simulink model "sm_car_"  (R2026b)
settings: Solver=ode23t  StopTime=100  MaxStep=0.4  AbsTol=1e-3  EnableMultiTasking=on
PreLoadFcn:
  | % Due to usability issue in Repeating Sequence block
  | warning('off','Simulink:Masking:Invalid');
  | 
  | % Eliminate unnecessary warnings in inactive variants
  | % Warnings generated only if you click through inactive variant
  | warning('off','MATLAB:nonExistentField');
  | warning('off','Simulink:Parameters:BlkParamUndefined');
PostLoadFcn:
  | set_param([bdroot '/Vehicle'],'popup_trailer','Off')
  | warning('off','sm:sli:setup:compile:LocalSolverNotSupported')
  | %sm_car_config_maneuver(bdroot,'WOT Braking');
  | sm_car_config_vehicle(bdroot,'false');
  | sm_car_config_logging(bdroot);
InitFcn:
  | sm_car_config_camera;
  | Vehicle = sm_car_vehcfg_checkConfig(Vehicle);
  | sm_car_check_tire_model(bdroot);
StartFcn:
  | tic;
StopFcn:
  | Elapsed_Sim_Time = toc;
  | % disp(['Elapsed Sim Time = ' num2str(Elapsed_Sim_Time)]);
undefined symbols (not defined in the file or in its folder): acc_theta, accel_ramp_rate, Axle1D, AxleIn, Camera, Control, Driver, Init, Maneuver, Pedal, Scene, ShaftL1, ShaftL2, ShaftR1, ShaftR2, Visual, X, xy_data_car_side, Y, Z
libraries: sm_lib x290, fl_lib x171, nesl_utility x144, simulink x60, simulink_extras x14, sdl_lib x14, SimscapeFluids_lib x7, Damper_Element x4, Tire_1x2x x4, ee_lib x3, Scene_Utilities x3, sharedTrackingLibrary x2
(part 9 of 22)

== system sm_car_/Controller/TrqVec_FLC/Brake Control/Pedal ==
  rBrakePedal : Inport
  VehBus : Inport  Port=2
  Apply{,1..3} (4 alike) : Constant  Value=[0 1]
  Bus Creator : BusCreator  Inputs=1
  Bus Creator1 : BusCreator  Inputs=4
  Terminator : Terminator
  Terminator1 : Terminator
  Brakes : Outport  VectorParamsAs1DForOutWhenUnconnected=off
  wires:
  rBrakePedal/1 -> Terminator1/1
  Apply3/1 -> Bus Creator1/4  "R2"
  Apply2/1 -> Bus Creator1/3  "L2"
  Apply1/1 -> Bus Creator1/2  "R1"
  Apply/1 -> Bus Creator1/1  "L1"
  Bus Creator1/1 -> Bus Creator/1  "Valves"
  VehBus/1 -> Terminator/1
  Bus Creator/1 -> Brakes/1  "Brakes"

== system sm_car_/Controller/TrqVec_FLC_V2/Brake Control/Pedal ==
  rBrakePedal : Inport
  VehBus : Inport  Port=2
  Apply{,1..3} (4 alike) : Constant  Value=[0 1]
  Bus Creator : BusCreator  Inputs=1
  Bus Creator1 : BusCreator  Inputs=4
  Terminator : Terminator
  Terminator1 : Terminator
  Brakes : Outport  VectorParamsAs1DForOutWhenUnconnected=off
  wires:
  Bus Creator/1 -> Brakes/1  "Brakes"
  VehBus/1 -> Terminator/1
  Bus Creator1/1 -> Bus Creator/1  "Valves"
  Apply/1 -> Bus Creator1/1  "L1"
  Apply1/1 -> Bus Creator1/2  "R1"
  Apply2/1 -> Bus Creator1/3  "L2"
  Apply3/1 -> Bus Creator1/4  "R2"
  rBrakePedal/1 -> Terminator1/1

== system sm_car_/Controller/TrqVec_FLC_V3/Brake Control/Pedal ==
  rBrakePedal : Inport
  VehBus : Inport  Port=2
  Apply{,1..3} (4 alike) : Constant  Value=[0 1]
  Bus Creator : BusCreator  Inputs=1
  Bus Creator1 : BusCreator  Inputs=4
  Terminator : Terminator
  Terminator1 : Terminator
  Brakes : Outport  VectorParamsAs1DForOutWhenUnconnected=off
  wires:
  rBrakePedal/1 -> Terminator1/1
  Apply3/1 -> Bus Creator1/4  "R2"
  Apply2/1 -> Bus Creator1/3  "L2"
  Apply1/1 -> Bus Creator1/2  "R1"
  Apply/1 -> Bus Creator1/1  "L1"
  Bus Creator1/1 -> Bus Creator/1  "Valves"
  VehBus/1 -> Terminator/1
  Bus Creator/1 -> Brakes/1  "Brakes"

== system sm_car_/Controller/TrqVec_FLC_V3/Power Control/State Estimation ==
  aSteerWheel : Inport
  VehBus : Inport  Port=2
  Bus Creator : BusCreator  Inputs=5
  Bus Selector : BusSelector  OutputSignals=World.vx,World.vy,World.vz,Chassis.Body.CG.nYaw,Chassis.Body.CG.gx,Chassis.Body.CG.gy,Chassis.SuspA1.LinkageL.Upright.Upright.w,Chassis.SuspA1.LinkageR.Upright.Upright.w,Chassis.SuspA2.LinkageL.Upright.Upright.w,Chassis.SuspA2.LinkageR.Upright.Upright.w
  Data Type Conversion : DataTypeConversion  OutDataTypeStr=double  SaturateOnIntegerOverflow=off  RndMeth=Floor
  Data Type Conversion1 : DataTypeConversion  OutDataTypeStr=double  SaturateOnIntegerOverflow=off  RndMeth=Floor
  Demux : Demux  Outputs=5
  Rate Transition1 : RateTransition  Deterministic=off  OutPortSampleTime=0.003
  Rate Transition2 : RateTransition  Deterministic=off  OutPortSampleTime=0.003
  Rate Transition4 : RateTransition  Deterministic=off
  Sensor Noise Simulation : Subsystem
  UKF : Subsystem
  StateEst : Outport
  Out Bus Element : Outport  Port=2  PortName=Meas  Element=Meas
  Out Bus Element1 : Outport  Port=2  PortName=Meas  Element=Input
  Out Bus Element2 : Outport  Port=2  PortName=Meas  Element=State
  wires:
  Bus Selector/3 -> Sensor Noise Simulation/3(<vz>)  "<vz>"
  Rate Transition4/1 -> Out Bus Element1/1
  Data Type Conversion1/1 -> Rate Transition4/1
  UKF/1(xhat) -> Data Type Conversion/1
  Rate Transition2/1 -> UKF/2(y1)
  Rate Transition1/1 -> UKF/1(StateTransitionFcnInputs)
  Demux/5 -> Bus Creator/5  "a_y"
  Demux/4 -> Bus Creator/4  "a_x"
  Demux/3 -> Bus Creator/3  "phi_dot"
  Demux/2 -> Bus Creator/2  "v_y"
  Demux/1 -> Bus Creator/1  "v_x"
  Bus Creator/1 -> StateEst/1, Out Bus Element2/1  "UKF"
  Data Type Conversion/1 -> Demux/1
  Sensor Noise Simulation/1(Inputs) -> Rate Transition1/1, Data Type Conversion1/1  "Input"
  Sensor Noise Simulation/2(Meas) -> Out Bus Element/1, Rate Transition2/1  "Measument"
  aSteerWheel/1 -> Sensor Noise Simulation/11(delta)  "delta"
  Bus Selector/10 -> Sensor Noise Simulation/10(<w_rr>)  "<w>"
  Bus Selector/9 -> Sensor Noise Simulation/9(<w_rl>)  "<w>"
  Bus Selector/8 -> Sensor Noise Simulation/8(<w_fr>)  "<w>"
  Bus Selector/7 -> Sensor Noise Simulation/7(<w_fl>)  "<w>"
  Bus Selector/6 -> Sensor Noise Simulation/6(<gy>)  "<gy>"
  Bus Selector/5 -> Sensor Noise Simulation/5(<gx>)  "<gx>"
  Bus Selector/4 -> Sensor Noise Simulation/4(<nYaw>)  "<nYaw>"
  Bus Selector/2 -> Sensor Noise Simulation/2(<vy>)  "<vy>"
  Bus Selector/1 -> Sensor Noise Simulation/1(<vx>)  "<vx>"
  VehBus/1 -> Bus Selector/1

== system sm_car_/Driver/Closed Loop/Driver/Get Pose ==
  Ref : Inport
  Bus Selector : BusSelector  OutputSignals=x,y,ayaw
  Gain : Gain  Gain=180/pi
  Mux : Mux  Inputs=3
  RefPose : Outport  VectorParamsAs1DForOutWhenUnconnected=off
  wires:
  Gain/1 -> Mux/3
  Bus Selector/3 -> Gain/1  "<ayaw>"
  Bus Selector/2 -> Mux/2  "<y>"
  Mux/1 -> RefPose/1
  Ref/1 -> Bus Selector/1
  Bus Selector/1 -> Mux/1  "<x>"

== system sm_car_/Driver/Closed Loop/Driver Override/None ==
  In : Inport
  DrvBus : Outport
  wires:
  In/1 -> DrvBus/1

== system sm_car_/Driver/Closed Loop/Driver Override/Override ==
  In : Inport
  Bus Creator5 : BusCreator  Inputs=4
  Bus Selector : BusSelector  OutputSignals=Reference,aSteerWheel,rAccelPedal,rBrakePedal
  Clock : Clock
  Compare To Constant : simulink/Logic and Bit Operations/Compare To Constant  relop=>=  const=Maneuver.TStart.aSteer.Value  OutDataTypeStr=boolean
  Compare To Constant1 : simulink/Logic and Bit Operations/Compare To Constant  relop=>=  const=Maneuver.TStart.rAccel.Value  OutDataTypeStr=boolean
  Compare To Constant2 : simulink/Logic and Bit Operations/Compare To Constant  relop=>=  const=Maneuver.TStart.rBrake.Value  OutDataTypeStr=boolean
  Input Sequence Accel Pedal : simulink/Sources/Repeating Sequence  rep_seq_t=Maneuver.Accel.t.Value  rep_seq_y=Maneuver.Accel.rPedal.Value
  Input Sequence Brake Pedal : simulink/Sources/Repeating Sequence  rep_seq_t=Maneuver.Brake.t.Value  rep_seq_y=Maneuver.Brake.rPedal.Value
  Input Sequence Steering Wheel : simulink/Sources/Repeating Sequence  rep_seq_t=Maneuver.Steer.t.Value  rep_seq_y=Maneuver.Steer.aWheel.Value
  Switch : Switch  Criteria=u2 > Threshold  SaturateOnIntegerOverflow=off  InputSameDT=off
  Switch1 : Switch  Criteria=u2 > Threshold  SaturateOnIntegerOverflow=off  InputSameDT=off
  Switch2 : Switch  Criteria=u2 > Threshold  SaturateOnIntegerOverflow=off  InputSameDT=off
  DrvBus : Outport
  wires:
  Input Sequence Brake Pedal/1 -> Switch2/1  "rBrakePedal"
  Input Sequence Accel Pedal/1 -> Switch1/1  "rAccelPedal"
  Input Sequence Steering Wheel/1 -> Switch/1  "aSteerWheel"
  Switch2/1 -> Bus Creator5/4  "rBrakePedal"
  Compare To Constant/1 -> Switch/2
  Clock/1 -> Compare To Constant/1, Compare To Constant1/1, Compare To Constant2/1
  Bus Selector/4 -> Switch2/3  "<rBrakePedal>"
  Switch1/1 -> Bus Creator5/3  "rAccelPedal"
  Bus Selector/3 -> Switch1/3  "<rAccelPedal>"
  Bus Selector/1 -> Bus Creator5/1  "<Reference>"
  Switch/1 -> Bus Creator5/2  "aSteerWheel"
  Bus Selector/2 -> Switch/3  "<aSteerWheel>"
  Bus Creator5/1 -> DrvBus/1  "DrvBus"
  In/1 -> Bus Selector/1
  Compare To Constant1/1 -> Switch1/2
  Compare To Constant2/1 -> Switch2/2

== system sm_car_/Driver/Closed Loop/Maneuver/Count Lap ==
  note: If on the previous step, the vehicle was in the first 5 percent of the trajectory and now it is on the last 5 percent of the trajectory, decrement the number of laps.
  note: If on the previous step, the vehicle was in the last 5 percent of the trajectory and now it is on the first 5 percent of the trajectory, increment the number of laps.
  ad : Inport
  AND Add Lap : Logic  IconShape=distinctive  AllPortsSameDT=off  OutDataTypeStr=boolean
  AND Subtract Lap : Logic  IconShape=distinctive  AllPortsSameDT=off  OutDataTypeStr=boolean
  Data Type Conversion : DataTypeConversion  SaturateOnIntegerOverflow=off  RndMeth=Floor
  Data Type Conversion1 : DataTypeConversion  SaturateOnIntegerOverflow=off  RndMeth=Floor
  First 5 Percent : simulink/Logic and Bit Operations/Compare To Constant  relop=<=  const=max(Maneuver.Trajectory.xTrajectory.Value)*0.05  OutDataTypeStr=boolean  ZeroCross=off
  Last 5 Percent : simulink/Logic and Bit Operations/Compare To Constant  relop=>=  const=max(Maneuver.Trajectory.xTrajectory.Value)*0.95  OutDataTypeStr=boolean  ZeroCross=off
  Memory : Memory  InitialCondition=false
  Memory2 : Memory  InitialCondition=false
  OR : Logic  Operator=OR  IconShape=distinctive  AllPortsSameDT=off  OutDataTypeStr=boolean
  Sum : Sum  Inputs=+-|
  Triggered Subsystem : Subsystem  TreatAsAtomicUnit=on
  lapC : Outport  VectorParamsAs1DForOutWhenUnconnected=off
  wires:
  Sum/1 -> Triggered Subsystem/1(Up Down)  "Counter"
  AND Subtract Lap/1 -> Data Type Conversion1/1, OR/2  "Subtract Lap"
  AND Add Lap/1 -> OR/1, Data Type Conversion/1  "Add Lap"
  Memory2/1 -> AND Subtract Lap/1
  OR/1 -> Triggered Subsystem/Trigger  "Trigger"
  Memory/1 -> AND Add Lap/1
  First 5 Percent/1 -> AND Add Lap/2, Memory2/1  "First 5"
  Triggered Subsystem/1(Num Laps) -> lapC/1
  Last 5 Percent/1 -> Memory/1, AND Subtract Lap/2  "Last 5"
  ad/1 -> Last 5 Percent/1, First 5 Percent/1
  Data Type Conversion/1 -> Sum/1
  Data Type Conversion1/1 -> Sum/2

== system sm_car_/Driver/Closed Loop/Maneuver/PoseTargetVisual ==
  note: Allow yaw angle to wrap for
      | clockwise and counterclockwise laps.
  dist : Inport
  ref_x : Inport  Port=2
  ref_y : Inport  Port=3
  ref_z : Inport  Port=4
  ref_ayaw : Inport  Port=5
  CW or CCW : Constant  Value=sign(Maneuver.Trajectory.aYaw.Value(end)-Maneuver.Trajectory.aYaw.Value(1))
  Count Lap : Subsystem
  Gain : Gain  Gain=2*pi
  MechanismConfiguration : sm_lib/Utilities/Mechanism Configuration  UniformGravity=None  GravityVector=[0 0 -9.80665]  GravityVectorUnits=m/s^2  LinearizationDelta=0.001  JointModeTransitionNonlinearIterations=2
  Pace Car : Subsystem  mask(Car Body Geometry){whl_cutout_rad=0.5, whl_base=abs(Vehicle.Chassis.Body.sAxle1.Value(1)-Vehicle.Chassis.Body.sAxle2.Value(1)), thk_top=0.05, thk_side=0.05, car_track=Vehicle.Chassis.Body.Width.Value, offset_ref=[0 0 0.3225], extr_data_emblem_f=Visual.PaceCar.emblem.data*0.2, extr_data_emblem_r=Visual.PaceCar.emblem.data*0.2, clr_body_geo_top=Visual.PaceCar.body.clr, opc_body_geo_top=Visual.PaceCar.body.opc, clr_body_geo_left=Visual.PaceCar.body.clr, opc_body_geo_left=Visual.PaceCar.body.opc, clr_body_geo_right=Visual.PaceCar.body.clr, opc_body_geo_right=Visual.PaceCar.body.opc, clr_emblem_f=Visual.PaceCar.body.clr, opc_emblem_f=Visual.PaceCar.emblem.opc, clr_emblem_r=Visual.PaceCar.body.clr, opc_emblem_r=Visual.PaceCar.emblem.opc}
      mask prompts: whl_cutout_rad "Wheel Cutout Radius (m)"; whl_base "Wheelbase (m)"; thk_top "Top Thickness (m)"; thk_side "Side Thickness (m)"; car_track "Width (m)"; offset_ref "Offset to reference frame [xyz] (m)"; extr_data_emblem_f "Emblem Data Front [xy] (m)"; extr_data_emblem_r "Emblem Data Rear [xy] (m)"
      mask help: Creates simple car geometry. Adjusting the wheel cutout radius and wheelbase causes the profile to be adjusted. Press the Plot Profile button to see how the parameters affect the profile.
      mask init:
      | [xy_data_car_top xy_data_car_side] = Extr_Data_Car_Profile(whl_cutout_rad, whl_base,thk_top);
      mask TypeOptions extr_data_emblem_f:
      | Ornament
      | Front/ExtrusionCrossSection
      mask TypeOptions extr_data_emblem_r:
      | Ornament
      | Rear/ExtrusionCrossSection
      mask TypeOptions clr_body_geo_top: Top Surface/GraphicDiffuseColor
      mask TypeOptions opc_body_geo_top: Top Surface/GraphicOpacity
      mask TypeOptions clr_body_geo_left: Left Face/GraphicDiffuseColor
      mask TypeOptions opc_body_geo_left: Left Face/GraphicOpacity
      mask TypeOptions clr_body_geo_right: Right Face/GraphicDiffuseColor
      mask TypeOptions opc_body_geo_right: Right Face/GraphicOpacity
      mask TypeOptions clr_emblem_f:
      | Ornament
      | Front/GraphicDiffuseColor
      mask TypeOptions opc_emblem_f:
      | Ornament
      | Front/GraphicOpacity
      mask TypeOptions clr_emblem_r:
      | Ornament
      | Rear/GraphicDiffuseColor
      mask TypeOptions opc_emblem_r:
      | Ornament
      | Rear/GraphicOpacity
      mask DialogControl cont_geometry Prompt: Body Geometry
      mask DialogControl push_plot_profile Prompt: Plot Profile
      mask DialogControl push_plot_profile Callback:
      | v = get_param(gcb,'MaskWSVariables');
      | getMaskValue = containers.Map({v.Name}',{v.Value}');
      | evalin('base',...
      |     sprintf('Extr_Data_Car_Profile(%s,%s,%s,''%s'');',...
      |     num2str(getMaskValue('whl_cutout_rad')),...
      |     num2str(getMaskValue('whl_base')),...
      |     num2str(getMaskValue('thk_top')),'plot'));
      mask DialogControl cont_emblem Prompt: Emblem
      mask DialogControl cont_vis Prompt: Visualization
      mask DialogControl text_vis_clr Prompt: Color [RGB]
      mask DialogControl text_vis_opc Prompt: Opac. (0-1)
      mask DialogControl text_vis_top Prompt: Top
      mask DialogControl text_vis_left Prompt: Left Side
      mask DialogControl text_vis_right Prompt: Right Side
      mask DialogControl text_vis_emblem_f Prompt: Emblem Front
      mask DialogControl text_vis_emblem_r Prompt: Emblem Rear
      mask Display: image('sm_car_bodygeometry_sedan.png');
  Planar Joint : sm_lib/Joints/Planar Joint  JointMode=Normal  CompositeWrenchDir=FollowerOnBase  CompositeWrenchFrame=BaseFrame  SenseConstraintForce=off  SenseConstraintTorque=off  SenseTotalForce=off  SenseTotalTorque=off  PxPositionTargetSpecify=off  PxPositionTargetPriority=High  PxPositionTargetValue=0  PxPositionTargetValueUnits=m  PxVelocityTargetSpecify=off  PxVelocityTargetPriority=High  PxVelocityTargetValue=0  PxVelocityTargetValueUnits=m/s  PxEquilibriumPosition=0  PxEquilibriumPositionUnits=m  PxSpringStiffness=1  PxSpringStiffnessUnits=N/m  PxDampingCoefficient=1  PxDampingCoefficientUnits=N/(m/s)  PxLowerLimitSpecify=off  PxLowerLimitBound=-1  PxLowerLimitBoundUnits=m  PxLowerLimitStiffness=1e6  PxLowerLimitStiffnessUnits=N/m  PxLowerLimitDamping=1e3  PxLowerLimitDampingUnits=N/(m/s)  PxLowerLimitTransitionRegionWidth=1e-4  PxLowerLimitTransitionRegionWidthUnits=m  PxUpperLimitSpecify=off  PxUpperLimitBound=1  PxUpperLimitBoundUnits=m  PxUpperLimitStiffness=1e6  PxUpperLimitStiffnessUnits=N/m  PxUpperLimitDamping=1e3  PxUpperLimitDampingUnits=N/(m/s)  PxUpperLimitTransitionRegionWidth=1e-4  PxUpperLimitTransitionRegionWidthUnits=m  PxTorqueActuationMode=ComputedTorque  PxMotionActuationMode=InputMotion  PxSensePosition=off  PxSenseVelocity=off  PxSenseAcceleration=off  PxSenseTorqueForce=off  PxSenseLowerLimitTorqueForce=off  PxSenseUpperLimitTorqueForce=off  PyPositionTargetSpecify=off  PyPositionTargetPriority=High  PyPositionTargetValue=0  PyPositionTargetValueUnits=m  PyVelocityTargetSpecify=off  PyVelocityTargetPriority=High  PyVelocityTargetValue=0  PyVelocityTargetValueUnits=m/s  PyEquilibriumPosition=0  PyEquilibriumPositionUnits=m  PySpringStiffness=1  PySpringStiffnessUnits=N/m  PyDampingCoefficient=1  PyDampingCoefficientUnits=N/(m/s)  PyLowerLimitSpecify=off  PyLowerLimitBound=-1  PyLowerLimitBoundUnits=m  PyLowerLimitStiffness=1e6  PyLowerLimitStiffnessUnits=N/m  PyLowerLimitDamping=1e3  PyLowerLimitDampingUnits=N/(m/s)  PyLowerLimitTransitionRegionWidth=1e-4  PyLowerLimitTransitionRegionWidthUnits=m  PyUpperLimitSpecify=off  PyUpperLimitBound=1  PyUpperLimitBoundUnits=m  PyUpperLimitStiffness=1e6  PyUpperLimitStiffnessUnits=N/m  PyUpperLimitDamping=1e3  PyUpperLimitDampingUnits=N/(m/s)  PyUpperLimitTransitionRegionWidth=1e-4  PyUpperLimitTransitionRegionWidthUnits=m  PyTorqueActuationMode=ComputedTorque  PyMotionActuationMode=InputMotion  PySensePosition=off  PySenseVelocity=off  PySenseAcceleration=off  PySenseTorqueForce=off  PySenseLowerLimitTorqueForce=off  PySenseUpperLimitTorqueForce=off  RzPositionTargetSpecify=off  RzPositionTargetPriority=High  RzPositionTargetValue=0  RzPositionTargetValueUnits=deg  RzVelocityTargetSpecify=off  RzVelocityTargetPriority=High  RzVelocityTargetValue=0  RzVelocityTargetValueUnits=deg/s  RzEquilibriumPosition=0  RzEquilibriumPositionUnits=deg  RzSpringStiffness=1  RzSpringStiffnessUnits=N*m/deg  RzDampingCoefficient=1  RzDampingCoefficientUnits=N*m/(deg/s)  RzLowerLimitSpecify=off  RzLowerLimitBound=-90  RzLowerLimitBoundUnits=deg  RzLowerLimitStiffness=1e4  RzLowerLimitStiffnessUnits=N*m/deg  RzLowerLimitDamping=10  RzLowerLimitDampingUnits=N*m/(deg/s)  RzLowerLimitTransitionRegionWidth=0.1  RzLowerLimitTransitionRegionWidthUnits=deg  RzUpperLimitSpecify=off  RzUpperLimitBound=90  RzUpperLimitBoundUnits=deg  RzUpperLimitStiffness=1e4  RzUpperLimitStiffnessUnits=N*m/deg  RzUpperLimitDamping=10  RzUpperLimitDampingUnits=N*m/(deg/s)  RzUpperLimitTransitionRegionWidth=0.1  RzUpperLimitTransitionRegionWidthUnits=deg  RzTorqueActuationMode=ComputedTorque  RzMotionActuationMode=InputMotion  RzSensePosition=off  RzSenseVelocity=off  RzSenseAcceleration=off  RzSenseTorqueForce=off  RzSenseLowerLimitTorqueForce=off  RzSenseUpperLimitTorqueForce=off
  Prismatic Joint : sm_lib/Joints/Prismatic Joint  JointMode=Normal  CompositeWrenchDir=FollowerOnBase  CompositeWrenchFrame=BaseFrame  SenseConstraintForce=off  SenseConstraintTorque=off  SenseTotalForce=off  SenseTotalTorque=off  PositionTargetSpecify=off  PositionTargetPriority=High  PositionTargetValue=0  PositionTargetValueUnits=m  VelocityTargetSpecify=off  VelocityTargetPriority=High  VelocityTargetValue=0  VelocityTargetValueUnits=m/s  EquilibriumPosition=0  EquilibriumPositionUnits=m  SpringStiffness=0  SpringStiffnessUnits=N/m  DampingCoefficient=0  DampingCoefficientUnits=N/(m/s)  LowerLimitSpecify=off  LowerLimitBound=-1  LowerLimitBoundUnits=m  LowerLimitStiffness=1e6  LowerLimitStiffnessUnits=N/m  LowerLimitDamping=1e3  LowerLimitDampingUnits=N/(m/s)  LowerLimitTransitionRegionWidth=1e-4  LowerLimitTransitionRegionWidthUnits=m  UpperLimitSpecify=off  UpperLimitBound=1  UpperLimitBoundUnits=m  UpperLimitStiffness=1e6  UpperLimitStiffnessUnits=N/m  UpperLimitDamping=1e3  UpperLimitDampingUnits=N/(m/s)  UpperLimitTransitionRegionWidth=1e-4  UpperLimitTransitionRegionWidthUnits=m  TorqueActuationMode=ComputedTorque  MotionActuationMode=InputMotion  SensePosition=off  SenseVelocity=off  SenseAcceleration=off  SenseTorqueForce=off  SenseLowerLimitTorqueForce=off  SenseUpperLimitTorqueForce=off
  Product : Product
  Rigid Transform : sm_lib/Frames and Transforms/Rigid Transform  RotationMethod=None  FollAlignAxisA=+X  BaseAlignAxisA=+Y  FollAlignAxisB=+Y  BaseAlignAxisB=+Z  RotationStandardAxis=+Z  RotationAngle=0.0  RotationAngleUnits=deg  RotationArbitraryAxis=[0 0 1]  RotationSequenceAxes=FollowerAxes  RotationSequence=XYX  RotationSequenceAngles=[0 0 0]  RotationSequenceAnglesUnits=deg  RotationMatrix=[1 0 0; 0 1 0; 0 0 1]  Quaternion=[1 0 0 0]  TranslationMethod=Cartesian  TranslationCartesianOffset=[0 0 0.1]  TranslationCartesianOffsetUnits=m  TranslationStandardAxis=+Z  TranslationStandardOffset=0  TranslationStandardOffsetUnits=m  TranslationROffset=0  TranslationROffsetUnits=m  TranslationThetaOffset=0  TranslationThetaOffsetUnits=deg  TranslationZOffset=0  TranslationZOffsetUnits=m
  Simulink-PS Converter : nesl_utility/Simulink-PS Converter  PhysicalDomain=network_engine_domain  SubClassName=ps_input  LeftPortType=input  RightPortType=output  PseudoPeriodic=off  Frequencies=[]  NoiseDistribution=none  NoiseParameters=[]  Unit=1  AffineConversion=off  FilteringAndDerivatives=filter  SimscapeFilterOrder=2  InputFilterTimeConstant=0.1  UdotUserProvided=0
  Simulink-PS Converter1 : nesl_utility/Simulink-PS Converter  PhysicalDomain=network_engine_domain  SubClassName=ps_input  LeftPortType=input  RightPortType=output  PseudoPeriodic=off  Frequencies=[]  NoiseDistribution=none  NoiseParameters=[]  Unit=1  AffineConversion=off  FilteringAndDerivatives=filter  SimscapeFilterOrder=2  InputFilterTimeConstant=0.1  UdotUserProvided=0
  Simulink-PS Converter2 : nesl_utility/Simulink-PS Converter  PhysicalDomain=network_engine_domain  SubClassName=ps_input  LeftPortType=input  RightPortType=output  PseudoPeriodic=off  Frequencies=[]  NoiseDistribution=none  NoiseParameters=[]  Unit=rad  AffineConversion=off  FilteringAndDerivatives=filter  SimscapeFilterOrder=2  InputFilterTimeConstant=0.1  UdotUserProvided=0
  Simulink-PS Converter3 : nesl_utility/Simulink-PS Converter  PhysicalDomain=network_engine_domain  SubClassName=ps_input  LeftPortType=input  RightPortType=output  PseudoPeriodic=off  Frequencies=[]  NoiseDistribution=none  NoiseParameters=[]  Unit=1  AffineConversion=off  FilteringAndDerivatives=filter  SimscapeFilterOrder=2  InputFilterTimeConstant=0.1  UdotUserProvided=0
  Solver Configuration : nesl_utility/Solver Configuration  PhysicalDomain=network_engine_domain  SubClassName=solver  LeftPortType=input  RightPortType=generic  Tones=[]  Harmonics=[]  SimulateNoise=off  Profile=off  UseLocalSampling=off  EnableSwitchedLinearOptims=on  FrequencyDomain=off  UseCCode=off  RelTol=0.001  AbsTol=1e-06  MinStep=1e-09  ToWorkspace=off  RevertToSquareIcSolve=off  NumHomotopyIterations=100  PhasorMode=off  PhasorModeNumHarmonics=1  ConsistencySolver=NEWTON_XTOL_AFTER_FTOL  CanonicalOrdering=UNORDERED  OptimizeIntermediates=UNOPTIMIZED  MulticoreSolverChoice=BACKWARD_EULER  IndexReductionMethod=DerivativeReplacement  DoDC=off  ResidualTolerance=1e-9  ConsistencyTolSource=GLOBAL  ConsistencyAbsTol=0.001  ConsistencyRelTol=0.001  ConsistencyTolFactor=0.001  UseLocalSolver=off  LocalSolverChoice=NE_BACKWARD_EULER_ADVANCER  ResolveIndetEquations=on  FunctionEvalNumThread=1  LocalSolverSampleTime=0.001  DoFixedCost=off  MaxNonlinIter=5  MaxModeIter=2  ComputeImpulses=off  ImpulseIterations=2  LinearAlgebra=Sparse  LinearAlgebraNumThread=0  EquationFormulation=NE_TIME_EF  DelaysMemoryBudget=1024  AutomaticFiltering=on  FilteringTimeConstant=0.001  PartitionStorageMethod=AS_NEEDED  PartitionMemoryBudget=1024  PartitionMethod=FAST  MultibodyUseLocalSolver=off  MultibodyLocalSolverChoice=ODE1  MultibodyLocalSolverSampleTime=0.001
  Sum : Sum  Inputs=|++
  World Frame : sm_lib/Frames and Transforms/World Frame
  wires:
  ref_z/1 -> Simulink-PS Converter3/1
  ref_x/1 -> Simulink-PS Converter/1
  ref_y/1 -> Simulink-PS Converter1/1
  ref_ayaw/1 -> Sum/1
  dist/1 -> Count Lap/1(ad)  "ad"
  Count Lap/1(Lap Count) -> Gain/1
  Product/1 -> Sum/2
  Sum/1 -> Simulink-PS Converter2/1
  Gain/1 -> Product/1
  CW or CCW/1 -> Product/2
  connections:
  Simulink-PS Converter3/RConn1 -- Prismatic Joint/LConn2
  Prismatic Joint/LConn1 -- Planar Joint/RConn1
  Solver Configuration/RConn1 -- MechanismConfiguration/RConn1 -- Planar Joint/LConn1 -- World Frame/RConn1
  Simulink-PS Converter1/RConn1 -- Planar Joint/LConn3
  Rigid Transform/LConn1 -- Prismatic Joint/RConn1
  Simulink-PS Converter2/RConn1 -- Planar Joint/LConn4
  Simulink-PS Converter/RConn1 -- Planar Joint/LConn2
  Pace Car/LConn1 -- Rigid Transform/RConn1

== system sm_car_/Driver/Closed Loop/Maneuver/vx override ==
  note: Override speed signal using
      | gain (to set to zero) and/or with an
      | offset (for passing maneuver).
  vx : Inport
  Bus Selector2 : BusSelector  OutputSignals=offset,gain
  Constant5 : Constant  Value=Maneuver.Trajectory.vx.Value
  Product : Product
  Sum : Sum  Inputs=++|
  vx_ovr : Outport  VectorParamsAs1DForOutWhenUnconnected=off
  wires:
  vx/1 -> Bus Selector2/1
  Bus Selector2/2 -> Product/1  "<gain>"
  Sum/1 -> vx_ovr/1
  Constant5/1 -> Product/2
  Product/1 -> Sum/2
  Bus Selector2/1 -> Sum/1  "<offset>"

== system sm_car_/Driver/Closed Loop/Maneuver/x override ==
  note: Override speed signal using
      | gain (to set to zero) and/or with an
      | offset (for passing maneuver).
  x : Inport
  Bus Selector2 : BusSelector  OutputSignals=offset,gain
  Constant3 : Constant  Value=Maneuver.Trajectory.x.Value
  Product : Product
  Sum : Sum  Inputs=++|
  x_ovr : Outport  VectorParamsAs1DForOutWhenUnconnected=off
  wires:
  Bus Selector2/1 -> Sum/1  "<offset>"
  Product/1 -> Sum/2
  Constant3/1 -> Product/2
  Sum/1 -> x_ovr/1
  Bus Selector2/2 -> Product/1  "<gain>"
  x/1 -> Bus Selector2/1

== system sm_car_/Driver/Closed Loop/Maneuver/y override ==
  note: Override speed signal using
      | gain (to set to zero) and/or with an
      | offset (for passing maneuver).
  y : Inport
  Bus Selector2 : BusSelector  OutputSignals=offset,gain
  Constant4 : Constant  Value=Maneuver.Trajectory.y.Value
  Product : Product
  Sum : Sum  Inputs=++|
  y_ovr : Outport  VectorParamsAs1DForOutWhenUnconnected=off
  wires:
  y/1 -> Bus Selector2/1
  Bus Selector2/2 -> Product/1  "<gain>"
  Sum/1 -> y_ovr/1
  Constant4/1 -> Product/2
  Product/1 -> Sum/2
  Bus Selector2/1 -> Sum/1  "<offset>"

== system sm_car_/Driver/Closed Loop/Maneuver/z override ==
  note: Override speed signal using
      | gain (to set to zero) and/or with an
      | offset (for passing maneuver).
  z : Inport
  Bus Selector2 : BusSelector  OutputSignals=offset,gain
  Constant1 : Constant  Value=Maneuver.Trajectory.z.Value
  Product : Product
  Sum : Sum  Inputs=++|
  z_ovr : Outport  VectorParamsAs1DForOutWhenUnconnected=off
  wires:
  Bus Selector2/1 -> Sum/1  "<offset>"
  Product/1 -> Sum/2
  Constant1/1 -> Product/2
  Sum/1 -> z_ovr/1
  Bus Selector2/2 -> Product/1  "<gain>"
  z/1 -> Bus Selector2/1

== system sm_car_/Driver/Closed Loop/Override/None ==
  dist : Inport
  Obs : Inport  Port=2
  Bus Creator{,2..4} (4 alike) : BusCreator  Inputs=2
  Bus Creator1 : BusCreator  Inputs=4
  Constant{1..2,4,6} (4 alike) : Constant  Value=0
  Constant{3,5,7..8} (4 alike) : Constant
  Terminator : Terminator
  Terminator1 : Terminator
  Ovr : Outport  VectorParamsAs1DForOutWhenUnconnected=off
  wires:
  Bus Creator4/1 -> Bus Creator1/1  "x"
  Bus Creator/1 -> Bus Creator1/4  "vx"
  Bus Creator3/1 -> Bus Creator1/2  "y"
  Constant2/1 -> Bus Creator2/1  "offset"
  Bus Creator2/1 -> Bus Creator1/3  "z"
  Constant3/1 -> Bus Creator2/2  "gain"
  Constant4/1 -> Bus Creator3/1  "offset"
  Constant5/1 -> Bus Creator3/2  "gain"
  Constant7/1 -> Bus Creator4/2  "gain"
  Constant6/1 -> Bus Creator4/1  "offset"
  Constant8/1 -> Bus Creator/2  "gain"
  Constant1/1 -> Bus Creator/1  "offset"
  Bus Creator1/1 -> Ovr/1
  Obs/1 -> Terminator1/1
  dist/1 -> Terminator/1

== system sm_car_/Driver/Closed Loop1/Driver/Get Pose ==
  Ref : Inport
  Bus Selector : BusSelector  OutputSignals=x,y,ayaw
  Mux : Mux  Inputs=3
  RefPose : Outport  VectorParamsAs1DForOutWhenUnconnected=off
  wires:
  Bus Selector/1 -> Mux/1  "<x>"
  Ref/1 -> Bus Selector/1
  Mux/1 -> RefPose/1
  Bus Selector/2 -> Mux/2  "<y>"
  Bus Selector/3 -> Mux/3  "<ayaw>"

== system sm_car_/Driver/Closed Loop1/Driver/Trasform Pose ==
  CurPose : Inport
  Cos : Trigonometry  Operator=cos
  Cos1 : Trigonometry
  Demux : Demux  Outputs=3
  Gain : Gain  Gain=0.8232
  Gain1 : Gain  Gain=0.8232
  Gain2 : Gain  Gain=pi/180
  Mux : Mux  Inputs=3
  Subtract : Sum  Inputs=+-
  Subtract1 : Sum  Inputs=+-
  CurrPoseCG : Outport
  wires:
  Mux/1 -> CurrPoseCG/1
  Cos1/1 -> Gain1/1
  Gain/1 -> Subtract/2
  Subtract/1 -> Mux/1
  Subtract1/1 -> Mux/2
  Demux/2 -> Subtract1/1
  Demux/1 -> Subtract/1
  Cos/1 -> Gain/1
  Gain1/1 -> Subtract1/2
  Demux/3 -> Gain2/1
  Gain2/1 -> Cos/1, Cos1/1, Mux/3
  CurPose/1 -> Demux/1

== system sm_car_/Driver/Closed Loop1/Driver Override/None ==
  In : Inport
  DrvBus : Outport
  wires:
  In/1 -> DrvBus/1

== system sm_car_/Driver/Closed Loop1/Driver Override/Override ==
  In : Inport
  Bus Creator5 : BusCreator  Inputs=4
  Bus Selector : BusSelector  OutputSignals=Reference,aSteerWheel,rAccelPedal,rBrakePedal
  Clock : Clock
  Compare To Constant : simulink/Logic and Bit Operations/Compare To Constant  relop=>=  const=Maneuver.TStart.aSteer.Value  OutDataTypeStr=boolean
  Compare To Constant1 : simulink/Logic and Bit Operations/Compare To Constant  relop=>=  const=Maneuver.TStart.rAccel.Value  OutDataTypeStr=boolean
  Compare To Constant2 : simulink/Logic and Bit Operations/Compare To Constant  relop=>=  const=Maneuver.TStart.rBrake.Value  OutDataTypeStr=boolean
  Input Sequence Accel Pedal : simulink/Sources/Repeating Sequence  rep_seq_t=Maneuver.Accel.t.Value  rep_seq_y=Maneuver.Accel.rPedal.Value
  Input Sequence Brake Pedal : simulink/Sources/Repeating Sequence  rep_seq_t=Maneuver.Brake.t.Value  rep_seq_y=Maneuver.Brake.rPedal.Value
  Input Sequence Steering Wheel : simulink/Sources/Repeating Sequence  rep_seq_t=Maneuver.Steer.t.Value  rep_seq_y=Maneuver.Steer.aWheel.Value
  Switch : Switch  Criteria=u2 > Threshold  SaturateOnIntegerOverflow=off  InputSameDT=off
  Switch1 : Switch  Criteria=u2 > Threshold  SaturateOnIntegerOverflow=off  InputSameDT=off
  Switch2 : Switch  Criteria=u2 > Threshold  SaturateOnIntegerOverflow=off  InputSameDT=off
  DrvBus : Outport
  wires:
  Compare To Constant2/1 -> Switch2/2
  Compare To Constant1/1 -> Switch1/2
  In/1 -> Bus Selector/1
  Bus Creator5/1 -> DrvBus/1  "DrvBus"
  Bus Selector/2 -> Switch/3  "<aSteerWheel>"
  Switch/1 -> Bus Creator5/2  "aSteerWheel"
  Bus Selector/1 -> Bus Creator5/1  "<Reference>"
  Bus Selector/3 -> Switch1/3  "<rAccelPedal>"
  Switch1/1 -> Bus Creator5/3  "rAccelPedal"
  Bus Selector/4 -> Switch2/3  "<rBrakePedal>"
  Clock/1 -> Compare To Constant2/1, Compare To Constant1/1, Compare To Constant/1
  Compare To Constant/1 -> Switch/2
  Switch2/1 -> Bus Creator5/4  "rBrakePedal"
  Input Sequence Steering Wheel/1 -> Switch/1  "aSteerWheel"
  Input Sequence Accel Pedal/1 -> Switch1/1  "rAccelPedal"
  Input Sequence Brake Pedal/1 -> Switch2/1  "rBrakePedal"

== system sm_car_/Driver/Closed Loop1/Maneuver/Count Lap ==
  note: If on the previous step, the vehicle was in the first 5 percent of the trajectory and now it is on the last 5 percent of the trajectory, decrement the number of laps.
  note: If on the previous step, the vehicle was in the last 5 percent of the trajectory and now it is on the first 5 percent of the trajectory, increment the number of laps.
  ad : Inport
  AND Add Lap : Logic  IconShape=distinctive  AllPortsSameDT=off  OutDataTypeStr=boolean
  AND Subtract Lap : Logic  IconShape=distinctive  AllPortsSameDT=off  OutDataTypeStr=boolean
  Data Type Conversion : DataTypeConversion  SaturateOnIntegerOverflow=off  RndMeth=Floor
  Data Type Conversion1 : DataTypeConversion  SaturateOnIntegerOverflow=off  RndMeth=Floor
  First 5 Percent : simulink/Logic and Bit Operations/Compare To Constant  relop=<=  const=max(Maneuver.Trajectory.xTrajectory.Value)*0.05  OutDataTypeStr=boolean  ZeroCross=off
  Last 5 Percent : simulink/Logic and Bit Operations/Compare To Constant  relop=>=  const=max(Maneuver.Trajectory.xTrajectory.Value)*0.95  OutDataTypeStr=boolean  ZeroCross=off
  Memory : Memory  InitialCondition=false
  Memory2 : Memory  InitialCondition=false
  OR : Logic  Operator=OR  IconShape=distinctive  AllPortsSameDT=off  OutDataTypeStr=boolean
  Sum : Sum  Inputs=+-|
  Triggered Subsystem : Subsystem  TreatAsAtomicUnit=on
  lapC : Outport  VectorParamsAs1DForOutWhenUnconnected=off
  wires:
  Sum/1 -> Triggered Subsystem/1(Up Down)  "Counter"
  AND Subtract Lap/1 -> Data Type Conversion1/1, OR/2  "Subtract Lap"
  AND Add Lap/1 -> OR/1, Data Type Conversion/1  "Add Lap"
  Memory2/1 -> AND Subtract Lap/1
  OR/1 -> Triggered Subsystem/Trigger  "Trigger"
  Memory/1 -> AND Add Lap/1
  First 5 Percent/1 -> AND Add Lap/2, Memory2/1  "First 5"
  Triggered Subsystem/1(Num Laps) -> lapC/1
  Last 5 Percent/1 -> Memory/1, AND Subtract Lap/2  "Last 5"
  ad/1 -> Last 5 Percent/1, First 5 Percent/1
  Data Type Conversion/1 -> Sum/1
  Data Type Conversion1/1 -> Sum/2

== system sm_car_/Driver/Closed Loop1/Maneuver/PoseTarget Visual ==
  note: Allow yaw angle to wrap for
      | clockwise and counterclockwise laps.
  ref_z : Inport
  ref_y : Inport  Port=2
  ref_x : Inport  Port=3
  Lap Count : Inport  Port=4
  ref_ayaw : Inport  Port=5
  CW or CCW : Constant  Value=sign(Maneuver.Trajectory.aYaw.Value(end)-Maneuver.Trajectory.aYaw.Value(1))
  Gain : Gain  Gain=2*pi
  MechanismConfiguration : sm_lib/Utilities/Mechanism Configuration  UniformGravity=None  GravityVector=[0 0 -9.80665]  GravityVectorUnits=m/s^2  LinearizationDelta=0.001  JointModeTransitionNonlinearIterations=2
  Pace Car : Subsystem  mask(Car Body Geometry){whl_cutout_rad=0.5, whl_base=abs(Vehicle.Chassis.Body.sAxle1.Value(1)-Vehicle.Chassis.Body.sAxle2.Value(1)), thk_top=0.05, thk_side=0.05, car_track=Vehicle.Chassis.Body.Width.Value, offset_ref=[0 0 0.3225], extr_data_emblem_f=Visual.PaceCar.emblem.data*0.2, extr_data_emblem_r=Visual.PaceCar.emblem.data*0.2, clr_body_geo_top=Visual.PaceCar.body.clr, opc_body_geo_top=Visual.PaceCar.body.opc, clr_body_geo_left=Visual.PaceCar.body.clr, opc_body_geo_left=Visual.PaceCar.body.opc, clr_body_geo_right=Visual.PaceCar.body.clr, opc_body_geo_right=Visual.PaceCar.body.opc, clr_emblem_f=Visual.PaceCar.body.clr, opc_emblem_f=Visual.PaceCar.emblem.opc, clr_emblem_r=Visual.PaceCar.body.clr, opc_emblem_r=Visual.PaceCar.emblem.opc}
      mask prompts: whl_cutout_rad "Wheel Cutout Radius (m)"; whl_base "Wheelbase (m)"; thk_top "Top Thickness (m)"; thk_side "Side Thickness (m)"; car_track "Width (m)"; offset_ref "Offset to reference frame [xyz] (m)"; extr_data_emblem_f "Emblem Data Front [xy] (m)"; extr_data_emblem_r "Emblem Data Rear [xy] (m)"
      mask help: Creates simple car geometry. Adjusting the wheel cutout radius and wheelbase causes the profile to be adjusted. Press the Plot Profile button to see how the parameters affect the profile.
      mask init:
      | [xy_data_car_top xy_data_car_side] = Extr_Data_Car_Profile(whl_cutout_rad, whl_base,thk_top);
      mask TypeOptions extr_data_emblem_f:
      | Ornament
      | Front/ExtrusionCrossSection
      mask TypeOptions extr_data_emblem_r:
      | Ornament
      | Rear/ExtrusionCrossSection
      mask TypeOptions clr_body_geo_top: Top Surface/GraphicDiffuseColor
      mask TypeOptions opc_body_geo_top: Top Surface/GraphicOpacity
      mask TypeOptions clr_body_geo_left: Left Face/GraphicDiffuseColor
      mask TypeOptions opc_body_geo_left: Left Face/GraphicOpacity
      mask TypeOptions clr_body_geo_right: Right Face/GraphicDiffuseColor
      mask TypeOptions opc_body_geo_right: Right Face/GraphicOpacity
      mask TypeOptions clr_emblem_f:
      | Ornament
      | Front/GraphicDiffuseColor
      mask TypeOptions opc_emblem_f:
      | Ornament
      | Front/GraphicOpacity
      mask TypeOptions clr_emblem_r:
      | Ornament
      | Rear/GraphicDiffuseColor
      mask TypeOptions opc_emblem_r:
      | Ornament
      | Rear/GraphicOpacity
      mask DialogControl cont_geometry Prompt: Body Geometry
      mask DialogControl push_plot_profile Prompt: Plot Profile
      mask DialogControl push_plot_profile Callback:
      | v = get_param(gcb,'MaskWSVariables');
      | getMaskValue = containers.Map({v.Name}',{v.Value}');
      | evalin('base',...
      |     sprintf('Extr_Data_Car_Profile(%s,%s,%s,''%s'');',...
      |     num2str(getMaskValue('whl_cutout_rad')),...
      |     num2str(getMaskValue('whl_base')),...
      |     num2str(getMaskValue('thk_top')),'plot'));
      mask DialogControl cont_emblem Prompt: Emblem
      mask DialogControl cont_vis Prompt: Visualization
      mask DialogControl text_vis_clr Prompt: Color [RGB]
      mask DialogControl text_vis_opc Prompt: Opac. (0-1)
      mask DialogControl text_vis_top Prompt: Top
      mask DialogControl text_vis_left Prompt: Left Side
      mask DialogControl text_vis_right Prompt: Right Side
      mask DialogControl text_vis_emblem_f Prompt: Emblem Front
      mask DialogControl text_vis_emblem_r Prompt: Emblem Rear
      mask Display: image('sm_car_bodygeometry_sedan.png');
  Planar Joint : sm_lib/Joints/Planar Joint  JointMode=Normal  CompositeWrenchDir=FollowerOnBase  CompositeWrenchFrame=BaseFrame  SenseConstraintForce=off  SenseConstraintTorque=off  SenseTotalForce=off  SenseTotalTorque=off  PxPositionTargetSpecify=off  PxPositionTargetPriority=High  PxPositionTargetValue=0  PxPositionTargetValueUnits=m  PxVelocityTargetSpecify=off  PxVelocityTargetPriority=High  PxVelocityTargetValue=0  PxVelocityTargetValueUnits=m/s  PxEquilibriumPosition=0  PxEquilibriumPositionUnits=m  PxSpringStiffness=1  PxSpringStiffnessUnits=N/m  PxDampingCoefficient=1  PxDampingCoefficientUnits=N/(m/s)  PxLowerLimitSpecify=off  PxLowerLimitBound=-1  PxLowerLimitBoundUnits=m  PxLowerLimitStiffness=1e6  PxLowerLimitStiffnessUnits=N/m  PxLowerLimitDamping=1e3  PxLowerLimitDampingUnits=N/(m/s)  PxLowerLimitTransitionRegionWidth=1e-4  PxLowerLimitTransitionRegionWidthUnits=m  PxUpperLimitSpecify=off  PxUpperLimitBound=1  PxUpperLimitBoundUnits=m  PxUpperLimitStiffness=1e6  PxUpperLimitStiffnessUnits=N/m  PxUpperLimitDamping=1e3  PxUpperLimitDampingUnits=N/(m/s)  PxUpperLimitTransitionRegionWidth=1e-4  PxUpperLimitTransitionRegionWidthUnits=m  PxTorqueActuationMode=ComputedTorque  PxMotionActuationMode=InputMotion  PxSensePosition=off  PxSenseVelocity=off  PxSenseAcceleration=off  PxSenseTorqueForce=off  PxSenseLowerLimitTorqueForce=off  PxSenseUpperLimitTorqueForce=off  PyPositionTargetSpecify=off  PyPositionTargetPriority=High  PyPositionTargetValue=0  PyPositionTargetValueUnits=m  PyVelocityTargetSpecify=off  PyVelocityTargetPriority=High  PyVelocityTargetValue=0  PyVelocityTargetValueUnits=m/s  PyEquilibriumPosition=0  PyEquilibriumPositionUnits=m  PySpringStiffness=1  PySpringStiffnessUnits=N/m  PyDampingCoefficient=1  PyDampingCoefficientUnits=N/(m/s)  PyLowerLimitSpecify=off  PyLowerLimitBound=-1  PyLowerLimitBoundUnits=m  PyLowerLimitStiffness=1e6  PyLowerLimitStiffnessUnits=N/m  PyLowerLimitDamping=1e3  PyLowerLimitDampingUnits=N/(m/s)  PyLowerLimitTransitionRegionWidth=1e-4  PyLowerLimitTransitionRegionWidthUnits=m  PyUpperLimitSpecify=off  PyUpperLimitBound=1  PyUpperLimitBoundUnits=m  PyUpperLimitStiffness=1e6  PyUpperLimitStiffnessUnits=N/m  PyUpperLimitDamping=1e3  PyUpperLimitDampingUnits=N/(m/s)  PyUpperLimitTransitionRegionWidth=1e-4  PyUpperLimitTransitionRegionWidthUnits=m  PyTorqueActuationMode=ComputedTorque  PyMotionActuationMode=InputMotion  PySensePosition=off  PySenseVelocity=off  PySenseAcceleration=off  PySenseTorqueForce=off  PySenseLowerLimitTorqueForce=off  PySenseUpperLimitTorqueForce=off  RzPositionTargetSpecify=off  RzPositionTargetPriority=High  RzPositionTargetValue=0  RzPositionTargetValueUnits=deg  RzVelocityTargetSpecify=off  RzVelocityTargetPriority=High  RzVelocityTargetValue=0  RzVelocityTargetValueUnits=deg/s  RzEquilibriumPosition=0  RzEquilibriumPositionUnits=deg  RzSpringStiffness=1  RzSpringStiffnessUnits=N*m/deg  RzDampingCoefficient=1  RzDampingCoefficientUnits=N*m/(deg/s)  RzLowerLimitSpecify=off  RzLowerLimitBound=-90  RzLowerLimitBoundUnits=deg  RzLowerLimitStiffness=1e4  RzLowerLimitStiffnessUnits=N*m/deg  RzLowerLimitDamping=10  RzLowerLimitDampingUnits=N*m/(deg/s)  RzLowerLimitTransitionRegionWidth=0.1  RzLowerLimitTransitionRegionWidthUnits=deg  RzUpperLimitSpecify=off  RzUpperLimitBound=90  RzUpperLimitBoundUnits=deg  RzUpperLimitStiffness=1e4  RzUpperLimitStiffnessUnits=N*m/deg  RzUpperLimitDamping=10  RzUpperLimitDampingUnits=N*m/(deg/s)  RzUpperLimitTransitionRegionWidth=0.1  RzUpperLimitTransitionRegionWidthUnits=deg  RzTorqueActuationMode=ComputedTorque  RzMotionActuationMode=InputMotion  RzSensePosition=off  RzSenseVelocity=off  RzSenseAcceleration=off  RzSenseTorqueForce=off  RzSenseLowerLimitTorqueForce=off  RzSenseUpperLimitTorqueForce=off
  Prismatic Joint : sm_lib/Joints/Prismatic Joint  JointMode=Normal  CompositeWrenchDir=FollowerOnBase  CompositeWrenchFrame=BaseFrame  SenseConstraintForce=off  SenseConstraintTorque=off  SenseTotalForce=off  SenseTotalTorque=off  PositionTargetSpecify=off  PositionTargetPriority=High  PositionTargetValue=0  PositionTargetValueUnits=m  VelocityTargetSpecify=off  VelocityTargetPriority=High  VelocityTargetValue=0  VelocityTargetValueUnits=m/s  EquilibriumPosition=0  EquilibriumPositionUnits=m  SpringStiffness=0  SpringStiffnessUnits=N/m  DampingCoefficient=0  DampingCoefficientUnits=N/(m/s)  LowerLimitSpecify=off  LowerLimitBound=-1  LowerLimitBoundUnits=m  LowerLimitStiffness=1e6  LowerLimitStiffnessUnits=N/m  LowerLimitDamping=1e3  LowerLimitDampingUnits=N/(m/s)  LowerLimitTransitionRegionWidth=1e-4  LowerLimitTransitionRegionWidthUnits=m  UpperLimitSpecify=off  UpperLimitBound=1  UpperLimitBoundUnits=m  UpperLimitStiffness=1e6  UpperLimitStiffnessUnits=N/m  UpperLimitDamping=1e3  UpperLimitDampingUnits=N/(m/s)  UpperLimitTransitionRegionWidth=1e-4  UpperLimitTransitionRegionWidthUnits=m  TorqueActuationMode=ComputedTorque  MotionActuationMode=InputMotion  SensePosition=off  SenseVelocity=off  SenseAcceleration=off  SenseTorqueForce=off  SenseLowerLimitTorqueForce=off  SenseUpperLimitTorqueForce=off
  Product : Product
  Rigid Transform : sm_lib/Frames and Transforms/Rigid Transform  RotationMethod=None  FollAlignAxisA=+X  BaseAlignAxisA=+Y  FollAlignAxisB=+Y  BaseAlignAxisB=+Z  RotationStandardAxis=+Z  RotationAngle=0.0  RotationAngleUnits=deg  RotationArbitraryAxis=[0 0 1]  RotationSequenceAxes=FollowerAxes  RotationSequence=XYX  RotationSequenceAngles=[0 0 0]  RotationSequenceAnglesUnits=deg  RotationMatrix=[1 0 0; 0 1 0; 0 0 1]  Quaternion=[1 0 0 0]  TranslationMethod=Cartesian  TranslationCartesianOffset=[0 0 0.1]  TranslationCartesianOffsetUnits=m  TranslationStandardAxis=+Z  TranslationStandardOffset=0  TranslationStandardOffsetUnits=m  TranslationROffset=0  TranslationROffsetUnits=m  TranslationThetaOffset=0  TranslationThetaOffsetUnits=deg  TranslationZOffset=0  TranslationZOffsetUnits=m
  Simulink-PS Converter : nesl_utility/Simulink-PS Converter  PhysicalDomain=network_engine_domain  SubClassName=ps_input  LeftPortType=input  RightPortType=output  PseudoPeriodic=off  Frequencies=[]  NoiseDistribution=none  NoiseParameters=[]  Unit=1  AffineConversion=off  FilteringAndDerivatives=filter  SimscapeFilterOrder=2  InputFilterTimeConstant=0.1  UdotUserProvided=0
  Simulink-PS Converter1 : nesl_utility/Simulink-PS Converter  PhysicalDomain=network_engine_domain  SubClassName=ps_input  LeftPortType=input  RightPortType=output  PseudoPeriodic=off  Frequencies=[]  NoiseDistribution=none  NoiseParameters=[]  Unit=1  AffineConversion=off  FilteringAndDerivatives=filter  SimscapeFilterOrder=2  InputFilterTimeConstant=0.1  UdotUserProvided=0
  Simulink-PS Converter2 : nesl_utility/Simulink-PS Converter  PhysicalDomain=network_engine_domain  SubClassName=ps_input  LeftPortType=input  RightPortType=output  PseudoPeriodic=off  Frequencies=[]  NoiseDistribution=none  NoiseParameters=[]  Unit=rad  AffineConversion=off  FilteringAndDerivatives=filter  SimscapeFilterOrder=2  InputFilterTimeConstant=0.1  UdotUserProvided=0
  Simulink-PS Converter3 : nesl_utility/Simulink-PS Converter  PhysicalDomain=network_engine_domain  SubClassName=ps_input  LeftPortType=input  RightPortType=output  PseudoPeriodic=off  Frequencies=[]  NoiseDistribution=none  NoiseParameters=[]  Unit=1  AffineConversion=off  FilteringAndDerivatives=filter  SimscapeFilterOrder=2  InputFilterTimeConstant=0.1  UdotUserProvided=0
  Solver Configuration : nesl_utility/Solver Configuration  PhysicalDomain=network_engine_domain  SubClassName=solver  LeftPortType=input  RightPortType=generic  Tones=[]  Harmonics=[]  SimulateNoise=off  Profile=off  UseLocalSampling=off  EnableSwitchedLinearOptims=on  FrequencyDomain=off  UseCCode=off  RelTol=0.001  AbsTol=1e-06  MinStep=1e-09  ToWorkspace=off  RevertToSquareIcSolve=off  NumHomotopyIterations=100  PhasorMode=off  PhasorModeNumHarmonics=1  ConsistencySolver=NEWTON_XTOL_AFTER_FTOL  CanonicalOrdering=CANONICAL  OptimizeIntermediates=OPTIMIZED  MulticoreSolverChoice=BACKWARD_EULER  IndexReductionMethod=DerivativeReplacement  DoDC=off  ResidualTolerance=1e-9  ConsistencyTolSource=GLOBAL  ConsistencyAbsTol=0.001  ConsistencyRelTol=0.001  ConsistencyTolFactor=0.001  UseLocalSolver=off  LocalSolverChoice=NE_BACKWARD_EULER_ADVANCER  ResolveIndetEquations=on  FunctionEvalNumThread=1  LocalSolverSampleTime=0.001  DoFixedCost=off  MaxNonlinIter=5  MaxModeIter=2  ComputeImpulses=off  ImpulseIterations=2  LinearAlgebra=Sparse  LinearAlgebraNumThread=0  EquationFormulation=NE_TIME_EF  DelaysMemoryBudget=1024  AutomaticFiltering=on  FilteringTimeConstant=0.001  PartitionStorageMethod=AS_NEEDED  PartitionMemoryBudget=1024  PartitionMethod=FAST  MultibodyUseLocalSolver=off  MultibodyLocalSolverChoice=ODE1  MultibodyLocalSolverSampleTime=0.001
  Sum : Sum  Inputs=|++
  World Frame : sm_lib/Frames and Transforms/World Frame
  wires:
  CW or CCW/1 -> Product/2
  Gain/1 -> Product/1
  Sum/1 -> Simulink-PS Converter2/1
  Product/1 -> Sum/2
  Lap Count/1 -> Gain/1
  ref_ayaw/1 -> Sum/1
  ref_y/1 -> Simulink-PS Converter1/1
  ref_x/1 -> Simulink-PS Converter/1
  ref_z/1 -> Simulink-PS Converter3/1
  connections:
  Pace Car/LConn1 -- Rigid Transform/RConn1
  Simulink-PS Converter/RConn1 -- Planar Joint/LConn2
  Simulink-PS Converter2/RConn1 -- Planar Joint/LConn4
  Rigid Transform/LConn1 -- Prismatic Joint/RConn1
  Simulink-PS Converter1/RConn1 -- Planar Joint/LConn3
  World Frame/RConn1 -- Planar Joint/LConn1 -- MechanismConfiguration/RConn1 -- Solver Configuration/RConn1
  Prismatic Joint/LConn1 -- Planar Joint/RConn1
  Simulink-PS Converter3/RConn1 -- Prismatic Joint/LConn2

== system sm_car_/Driver/Closed Loop1/Maneuver/vx override ==
  note: Override speed signal using
      | gain (to set to zero) and/or with an
      | offset (for passing maneuver).
  vx : Inport
  Bus Selector2 : BusSelector  OutputSignals=offset,gain
  Constant5 : Constant  Value=Maneuver.Trajectory.vx.Value
  Product : Product
  Sum : Sum  Inputs=++|
  vx_ovr : Outport  VectorParamsAs1DForOutWhenUnconnected=off
  wires:
  Bus Selector2/1 -> Sum/1  "<offset>"
  Product/1 -> Sum/2
  Constant5/1 -> Product/2
  Sum/1 -> vx_ovr/1
  Bus Selector2/2 -> Product/1  "<gain>"
  vx/1 -> Bus Selector2/1

== system sm_car_/Driver/Closed Loop1/Maneuver/x override ==
  note: Override speed signal using
      | gain (to set to zero) and/or with an
      | offset (for passing maneuver).
  x : Inport
  Bus Selector2 : BusSelector  OutputSignals=offset,gain
  Constant3 : Constant  Value=Maneuver.Trajectory.x.Value
  Product : Product
  Sum : Sum  Inputs=++|
  x_ovr : Outport  VectorParamsAs1DForOutWhenUnconnected=off
  wires:
  x/1 -> Bus Selector2/1
  Bus Selector2/2 -> Product/1  "<gain>"
  Sum/1 -> x_ovr/1
  Constant3/1 -> Product/2
  Product/1 -> Sum/2
  Bus Selector2/1 -> Sum/1  "<offset>"

== system sm_car_/Driver/Closed Loop1/Maneuver/y override ==
  note: Override speed signal using
      | gain (to set to zero) and/or with an
      | offset (for passing maneuver).
  y : Inport
  Bus Selector2 : BusSelector  OutputSignals=offset,gain
  Constant4 : Constant  Value=Maneuver.Trajectory.y.Value
  Product : Product
  Sum : Sum  Inputs=++|
  y_ovr : Outport  VectorParamsAs1DForOutWhenUnconnected=off
  wires:
  Bus Selector2/1 -> Sum/1  "<offset>"
  Product/1 -> Sum/2
  Constant4/1 -> Product/2
  Sum/1 -> y_ovr/1
  Bus Selector2/2 -> Product/1  "<gain>"
  y/1 -> Bus Selector2/1

== system sm_car_/Driver/Closed Loop1/Maneuver/z override ==
  note: Override speed signal using
      | gain (to set to zero) and/or with an
      | offset (for passing maneuver).
  z : Inport
  Bus Selector2 : BusSelector  OutputSignals=offset,gain
  Constant1 : Constant  Value=Maneuver.Trajectory.z.Value
  Product : Product
  Sum : Sum  Inputs=++|
  z_ovr : Outport  VectorParamsAs1DForOutWhenUnconnected=off
  wires:
  z/1 -> Bus Selector2/1
  Bus Selector2/2 -> Product/1  "<gain>"
  Sum/1 -> z_ovr/1
  Constant1/1 -> Product/2
  Product/1 -> Sum/2
  Bus Selector2/1 -> Sum/1  "<offset>"
